simulink model "voltage_to_current_signal"  (R2024a)
settings: Solver=VariableStepAuto  StartTime=0.0  StopTime=0.1  RelTol=1e-3
libraries: fl_lib x93, nesl_utility x24
settings Model: Creator=ltnbda  LastModifiedBy=ltnbda
settings RTWCC: GPUComputeCapability=3.5

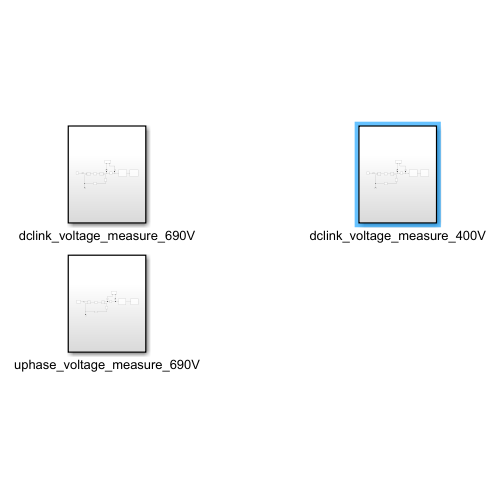
[thumbnail: Simulink's stored preview of the top-level diagram]
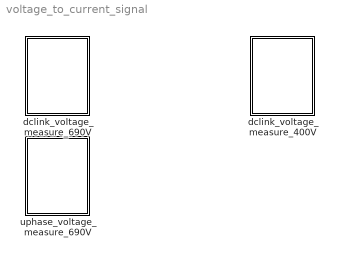
== system voltage_to_current_signal ==
  dclink_voltage_measure_400V : Subsystem
  dclink_voltage_measure_690V : Subsystem
  uphase_voltage_measure_690V : Subsystem

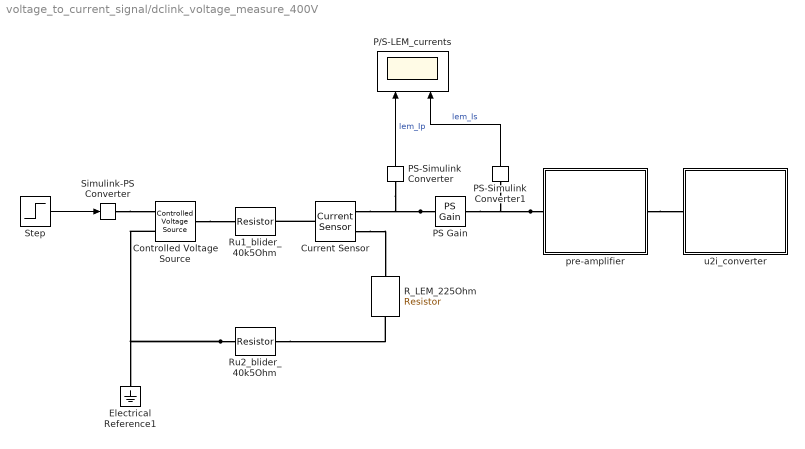
== system voltage_to_current_signal/dclink_voltage_measure_400V ==
  Controlled Voltage Source : fl_lib/Electrical/Electrical Sources/Controlled Voltage Source
  Current Sensor : fl_lib/Electrical/Electrical Sensors/Current Sensor
  Electrical Reference1 : fl_lib/Electrical/Electrical Elements/Electrical Reference
  P/S-LEM_currents : Scope  NumInputPorts=2
  PS Gain : fl_lib/Physical Signals/Functions/PS Gain  gain=2.5
  PS-Simulink Converter : nesl_utility/PS-Simulink Converter  PhysicalDomain=network_engine_domain  SubClassName=ps_output  LeftPortType=input  RightPortType=output  PseudoPeriodic=off  Frequencies=[]  VectorFormat=1-D array  Unit=A  AffineConversion=off
  PS-Simulink Converter1 : nesl_utility/PS-Simulink Converter  PhysicalDomain=network_engine_domain  SubClassName=ps_output  LeftPortType=input  RightPortType=output  PseudoPeriodic=off  Frequencies=[]  VectorFormat=1-D array  Unit=A  AffineConversion=off
  R_LEM_225Ohm : fl_lib/Electrical/Electrical Elements/Resistor  R=225 Ohm  i_specify=off  i_priority=None  i=0 A  i_nominal_specify=off  i_nominal_value=1  i_nominal_unit=A  v_specify=off  v_priority=None  v=0 V  v_nominal_specify=off  v_nominal_value=1  v_nominal_unit=V
  Ru1_blider_40k5Ohm : fl_lib/Electrical/Electrical Elements/Resistor  R=40.5e3 Ohm  i_specify=off  i_priority=None  i=0 A  i_nominal_specify=off  i_nominal_value=1  i_nominal_unit=A  v_specify=off  v_priority=None  v=0 V  v_nominal_specify=off  v_nominal_value=1  v_nominal_unit=V
  Ru2_blider_40k5Ohm : fl_lib/Electrical/Electrical Elements/Resistor  R=40.5e3 Ohm  i_specify=off  i_priority=None  i=0 A  i_nominal_specify=off  i_nominal_value=1  i_nominal_unit=A  v_specify=off  v_priority=None  v=0 V  v_nominal_specify=off  v_nominal_value=1  v_nominal_unit=V
  Simulink-PS Converter : nesl_utility/Simulink-PS Converter  PhysicalDomain=network_engine_domain  SubClassName=ps_input  LeftPortType=input  RightPortType=output  PseudoPeriodic=off  Frequencies=[]  NoiseDistribution=none  NoiseParameters=[]  Unit=V  AffineConversion=off  FilteringAndDerivatives=provide  SimscapeFilterOrder=1  InputFilterTimeConstant=0.001  UdotUserProvided=0
  Step : Step  Time=0.02  After=1000  SampleTime=0
  pre-amplifier : Subsystem
  u2i_converter : Subsystem
  wires:
  PS-Simulink Converter1/1 -> P/S-LEM_currents/2  "lem_Is"
  PS-Simulink Converter/1 -> P/S-LEM_currents/1  "lem_Ip"
  Step/1 -> Simulink-PS Converter/1
  connections:
  PS Gain/LConn1 -- PS-Simulink Converter/LConn1 -- Current Sensor/RConn1
  pre-amplifier/RConn1 -- u2i_converter/LConn1
  pre-amplifier/LConn1 -- PS-Simulink Converter1/LConn1 -- PS Gain/RConn1
  Current Sensor/RConn2 -- R_LEM_225Ohm/LConn1
  Current Sensor/LConn1 -- Ru1_blider_40k5Ohm/RConn1
  Ru2_blider_40k5Ohm/LConn1 -- Electrical Reference1/LConn1 -- Controlled Voltage Source/RConn2
  Controlled Voltage Source/LConn1 -- Ru1_blider_40k5Ohm/LConn1
  Ru2_blider_40k5Ohm/RConn1 -- R_LEM_225Ohm/RConn1
  Simulink-PS Converter/RConn1 -- Controlled Voltage Source/RConn1

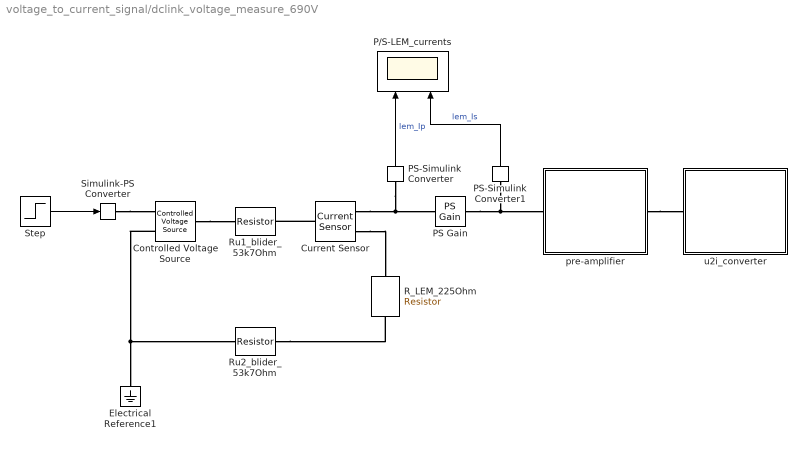
== system voltage_to_current_signal/dclink_voltage_measure_690V ==
  Controlled Voltage Source : fl_lib/Electrical/Electrical Sources/Controlled Voltage Source
  Current Sensor : fl_lib/Electrical/Electrical Sensors/Current Sensor
  Electrical Reference1 : fl_lib/Electrical/Electrical Elements/Electrical Reference
  P/S-LEM_currents : Scope  NumInputPorts=2
  PS Gain : fl_lib/Physical Signals/Functions/PS Gain  gain=2.5
  PS-Simulink Converter : nesl_utility/PS-Simulink Converter  PhysicalDomain=network_engine_domain  SubClassName=ps_output  LeftPortType=input  RightPortType=output  PseudoPeriodic=off  Frequencies=[]  VectorFormat=1-D array  Unit=A  AffineConversion=off
  PS-Simulink Converter1 : nesl_utility/PS-Simulink Converter  PhysicalDomain=network_engine_domain  SubClassName=ps_output  LeftPortType=input  RightPortType=output  PseudoPeriodic=off  Frequencies=[]  VectorFormat=1-D array  Unit=A  AffineConversion=off
  R_LEM_225Ohm : fl_lib/Electrical/Electrical Elements/Resistor  R=225 Ohm  i_specify=off  i_priority=None  i=0 A  i_nominal_specify=off  i_nominal_value=1  i_nominal_unit=A  v_specify=off  v_priority=None  v=0 V  v_nominal_specify=off  v_nominal_value=1  v_nominal_unit=V
  Ru1_blider_53k7Ohm : fl_lib/Electrical/Electrical Elements/Resistor  R=53.7e3 Ohm  i_specify=off  i_priority=None  i=0 A  i_nominal_specify=off  i_nominal_value=1  i_nominal_unit=A  v_specify=off  v_priority=None  v=0 V  v_nominal_specify=off  v_nominal_value=1  v_nominal_unit=V
  Ru2_blider_53k7Ohm : fl_lib/Electrical/Electrical Elements/Resistor  R=53.7e3 Ohm  i_specify=off  i_priority=None  i=0 A  i_nominal_specify=off  i_nominal_value=1  i_nominal_unit=A  v_specify=off  v_priority=None  v=0 V  v_nominal_specify=off  v_nominal_value=1  v_nominal_unit=V
  Simulink-PS Converter : nesl_utility/Simulink-PS Converter  PhysicalDomain=network_engine_domain  SubClassName=ps_input  LeftPortType=input  RightPortType=output  PseudoPeriodic=off  Frequencies=[]  NoiseDistribution=none  NoiseParameters=[]  Unit=V  AffineConversion=off  FilteringAndDerivatives=provide  SimscapeFilterOrder=1  InputFilterTimeConstant=0.001  UdotUserProvided=0
  Step : Step  Time=0.02  After=1500  SampleTime=0
  pre-amplifier : Subsystem
  u2i_converter : Subsystem
  wires:
  Step/1 -> Simulink-PS Converter/1
  PS-Simulink Converter/1 -> P/S-LEM_currents/1  "lem_Ip"
  PS-Simulink Converter1/1 -> P/S-LEM_currents/2  "lem_Is"
  connections:
  Simulink-PS Converter/RConn1 -- Controlled Voltage Source/RConn1
  Ru2_blider_53k7Ohm/RConn1 -- R_LEM_225Ohm/RConn1
  Controlled Voltage Source/LConn1 -- Ru1_blider_53k7Ohm/LConn1
  Controlled Voltage Source/RConn2 -- Electrical Reference1/LConn1 -- Ru2_blider_53k7Ohm/LConn1
  Current Sensor/LConn1 -- Ru1_blider_53k7Ohm/RConn1
  Current Sensor/RConn2 -- R_LEM_225Ohm/LConn1
  PS Gain/RConn1 -- PS-Simulink Converter1/LConn1 -- pre-amplifier/LConn1
  pre-amplifier/RConn1 -- u2i_converter/LConn1
  Current Sensor/RConn1 -- PS-Simulink Converter/LConn1 -- PS Gain/LConn1

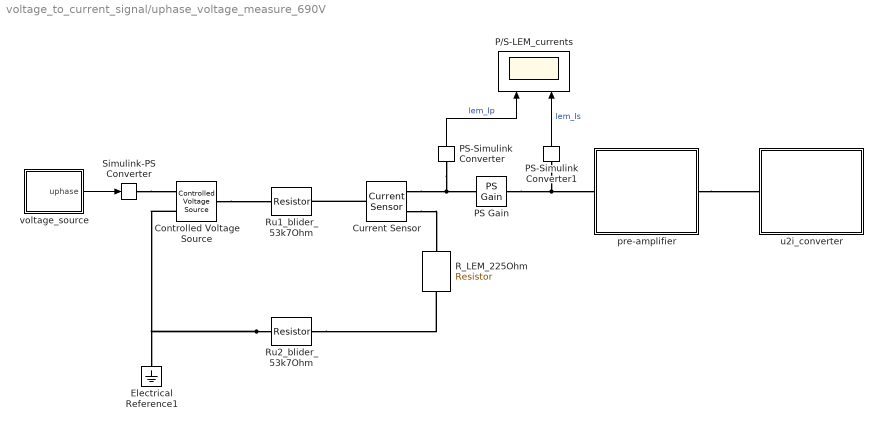
== system voltage_to_current_signal/uphase_voltage_measure_690V ==
  Controlled Voltage Source : fl_lib/Electrical/Electrical Sources/Controlled Voltage Source
  Current Sensor : fl_lib/Electrical/Electrical Sensors/Current Sensor
  Electrical Reference1 : fl_lib/Electrical/Electrical Elements/Electrical Reference
  P/S-LEM_currents : Scope  NumInputPorts=2
  PS Gain : fl_lib/Physical Signals/Functions/PS Gain  gain=2.5
  PS-Simulink Converter : nesl_utility/PS-Simulink Converter  PhysicalDomain=network_engine_domain  SubClassName=ps_output  LeftPortType=input  RightPortType=output  PseudoPeriodic=off  Frequencies=[]  VectorFormat=1-D array  Unit=A  AffineConversion=off
  PS-Simulink Converter1 : nesl_utility/PS-Simulink Converter  PhysicalDomain=network_engine_domain  SubClassName=ps_output  LeftPortType=input  RightPortType=output  PseudoPeriodic=off  Frequencies=[]  VectorFormat=1-D array  Unit=A  AffineConversion=off
  R_LEM_225Ohm : fl_lib/Electrical/Electrical Elements/Resistor  R=225 Ohm  i_specify=off  i_priority=None  i=0 A  i_nominal_specify=off  i_nominal_value=1  i_nominal_unit=A  v_specify=off  v_priority=None  v=0 V  v_nominal_specify=off  v_nominal_value=1  v_nominal_unit=V
  Ru1_blider_53k7Ohm : fl_lib/Electrical/Electrical Elements/Resistor  R=53.7e3 Ohm  i_specify=off  i_priority=None  i=0 A  i_nominal_specify=off  i_nominal_value=1  i_nominal_unit=A  v_specify=off  v_priority=None  v=0 V  v_nominal_specify=off  v_nominal_value=1  v_nominal_unit=V
  Ru2_blider_53k7Ohm : fl_lib/Electrical/Electrical Elements/Resistor  R=53.7e3 Ohm  i_specify=off  i_priority=None  i=0 A  i_nominal_specify=off  i_nominal_value=1  i_nominal_unit=A  v_specify=off  v_priority=None  v=0 V  v_nominal_specify=off  v_nominal_value=1  v_nominal_unit=V
  Simulink-PS Converter : nesl_utility/Simulink-PS Converter  PhysicalDomain=network_engine_domain  SubClassName=ps_input  LeftPortType=input  RightPortType=output  PseudoPeriodic=off  Frequencies=[]  NoiseDistribution=none  NoiseParameters=[]  Unit=V  AffineConversion=off  FilteringAndDerivatives=provide  SimscapeFilterOrder=1  InputFilterTimeConstant=0.001  UdotUserProvided=0
  pre-amplifier : Subsystem
  u2i_converter : Subsystem
  voltage_source : Subsystem
  wires:
  PS-Simulink Converter1/1 -> P/S-LEM_currents/2  "lem_Is"
  PS-Simulink Converter/1 -> P/S-LEM_currents/1  "lem_Ip"
  voltage_source/1(uphase) -> Simulink-PS Converter/1
  connections:
  PS-Simulink Converter/LConn1 -- Current Sensor/RConn1 -- PS Gain/LConn1
  pre-amplifier/RConn1 -- u2i_converter/LConn1
  PS-Simulink Converter1/LConn1 -- PS Gain/RConn1 -- pre-amplifier/LConn1
  Current Sensor/RConn2 -- R_LEM_225Ohm/LConn1
  Current Sensor/LConn1 -- Ru1_blider_53k7Ohm/RConn1
  Ru2_blider_53k7Ohm/LConn1 -- Electrical Reference1/LConn1 -- Controlled Voltage Source/RConn2
  Controlled Voltage Source/LConn1 -- Ru1_blider_53k7Ohm/LConn1
  Ru2_blider_53k7Ohm/RConn1 -- R_LEM_225Ohm/RConn1
  Simulink-PS Converter/RConn1 -- Controlled Voltage Source/RConn1

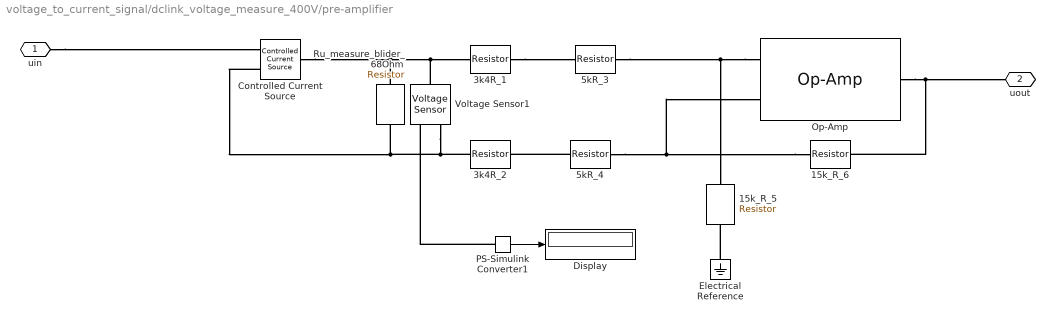
== system voltage_to_current_signal/dclink_voltage_measure_400V/pre-amplifier ==
  15k_R_5 : fl_lib/Electrical/Electrical Elements/Resistor  R=15e3 Ohm  i_specify=off  i_priority=None  i=0 A  i_nominal_specify=off  i_nominal_value=1  i_nominal_unit=A  v_specify=off  v_priority=None  v=0 V  v_nominal_specify=off  v_nominal_value=1  v_nominal_unit=V
  15k_R_6 : fl_lib/Electrical/Electrical Elements/Resistor  R=15e3 Ohm  i_specify=off  i_priority=None  i=0 A  i_nominal_specify=off  i_nominal_value=1  i_nominal_unit=A  v_specify=off  v_priority=None  v=0 V  v_nominal_specify=off  v_nominal_value=1  v_nominal_unit=V
  3k4R_1 : fl_lib/Electrical/Electrical Elements/Resistor  R=3.4e3 Ohm  i_specify=off  i_priority=None  i=0 A  i_nominal_specify=off  i_nominal_value=1  i_nominal_unit=A  v_specify=off  v_priority=None  v=0 V  v_nominal_specify=off  v_nominal_value=1  v_nominal_unit=V
  3k4R_2 : fl_lib/Electrical/Electrical Elements/Resistor  R=3.4e3 Ohm  i_specify=off  i_priority=None  i=0 A  i_nominal_specify=off  i_nominal_value=1  i_nominal_unit=A  v_specify=off  v_priority=None  v=0 V  v_nominal_specify=off  v_nominal_value=1  v_nominal_unit=V
  5kR_3 : fl_lib/Electrical/Electrical Elements/Resistor  R=5e3 Ohm  i_specify=off  i_priority=None  i=0 A  i_nominal_specify=off  i_nominal_value=1  i_nominal_unit=A  v_specify=off  v_priority=None  v=0 V  v_nominal_specify=off  v_nominal_value=1  v_nominal_unit=V
  5kR_4 : fl_lib/Electrical/Electrical Elements/Resistor  R=5e3 Ohm  i_specify=off  i_priority=None  i=0 A  i_nominal_specify=off  i_nominal_value=1  i_nominal_unit=A  v_specify=off  v_priority=None  v=0 V  v_nominal_specify=off  v_nominal_value=1  v_nominal_unit=V
  Controlled Current Source : fl_lib/Electrical/Electrical Sources/Controlled Current Source
  Display : Display
  Electrical Reference : fl_lib/Electrical/Electrical Elements/Electrical Reference
  Op-Amp : fl_lib/Electrical/Electrical Elements/Op-Amp  outI_specify=off  outI_priority=None  outI=0 A  outI_nominal_specify=off  outI_nominal_value=1  outI_nominal_unit=A
  PS-Simulink Converter1 : nesl_utility/PS-Simulink Converter  PhysicalDomain=network_engine_domain  SubClassName=ps_output  LeftPortType=input  RightPortType=output  PseudoPeriodic=off  Frequencies=[]  VectorFormat=1-D array  Unit=V  AffineConversion=off
  Ru_measure_blider_68Ohm : fl_lib/Electrical/Electrical Elements/Resistor  R=68 Ohm  i_specify=off  i_priority=None  i=0 A  i_nominal_specify=off  i_nominal_value=1  i_nominal_unit=A  v_specify=off  v_priority=None  v=0 V  v_nominal_specify=off  v_nominal_value=1  v_nominal_unit=V
  Voltage Sensor1 : fl_lib/Electrical/Electrical Sensors/Voltage Sensor
  uin : PMIOPort  Side=Left
  uout : PMIOPort  Port=2  Side=Right
  wires:
  PS-Simulink Converter1/1 -> Display/1
  connections:
  PS-Simulink Converter1/LConn1 -- Voltage Sensor1/RConn1
  uin/RConn1 -- Controlled Current Source/RConn1
  Ru_measure_blider_68Ohm/RConn1 -- Controlled Current Source/RConn2 -- Voltage Sensor1/RConn2 -- 3k4R_2/LConn1
  Controlled Current Source/LConn1 -- Voltage Sensor1/LConn1 -- 3k4R_1/LConn1 -- Ru_measure_blider_68Ohm/LConn1
  15k_R_6/LConn1 -- uout/RConn1 -- Op-Amp/RConn1
  15k_R_6/RConn1 -- Op-Amp/LConn2 -- 5kR_4/RConn1
  Op-Amp/LConn1 -- 15k_R_5/LConn1 -- 5kR_3/RConn1
  Electrical Reference/LConn1 -- 15k_R_5/RConn1
  5kR_4/LConn1 -- 3k4R_2/RConn1
  3k4R_1/RConn1 -- 5kR_3/LConn1

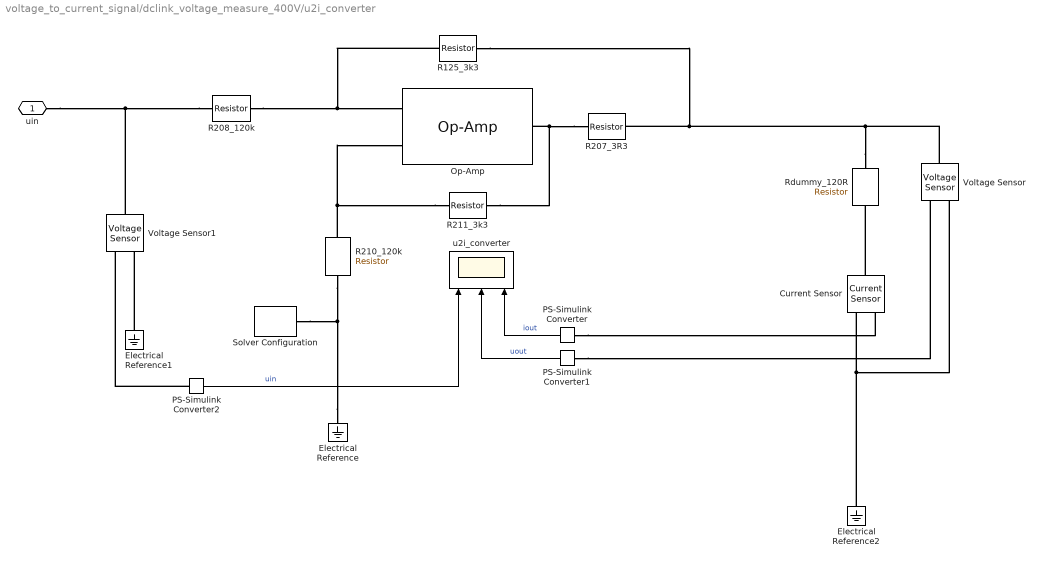
== system voltage_to_current_signal/dclink_voltage_measure_400V/u2i_converter ==
  Current Sensor : fl_lib/Electrical/Electrical Sensors/Current Sensor
  Electrical Reference : fl_lib/Electrical/Electrical Elements/Electrical Reference
  Electrical Reference1 : fl_lib/Electrical/Electrical Elements/Electrical Reference
  Electrical Reference2 : fl_lib/Electrical/Electrical Elements/Electrical Reference
  Op-Amp : fl_lib/Electrical/Electrical Elements/Op-Amp  outI_specify=off  outI_priority=None  outI=0 A  outI_nominal_specify=off  outI_nominal_value=1  outI_nominal_unit=A
  PS-Simulink Converter : nesl_utility/PS-Simulink Converter  PhysicalDomain=network_engine_domain  SubClassName=ps_output  LeftPortType=input  RightPortType=output  PseudoPeriodic=off  Frequencies=[]  VectorFormat=1-D array  Unit=A  AffineConversion=off
  PS-Simulink Converter1 : nesl_utility/PS-Simulink Converter  PhysicalDomain=network_engine_domain  SubClassName=ps_output  LeftPortType=input  RightPortType=output  PseudoPeriodic=off  Frequencies=[]  VectorFormat=1-D array  Unit=V  AffineConversion=off
  PS-Simulink Converter2 : nesl_utility/PS-Simulink Converter  PhysicalDomain=network_engine_domain  SubClassName=ps_output  LeftPortType=input  RightPortType=output  PseudoPeriodic=off  Frequencies=[]  VectorFormat=1-D array  Unit=V  AffineConversion=off
  R125_3k3 : fl_lib/Electrical/Electrical Elements/Resistor  R=3.3e3 Ohm  i_specify=off  i_priority=None  i=0 A  i_nominal_specify=off  i_nominal_value=1  i_nominal_unit=A  v_specify=off  v_priority=None  v=0 V  v_nominal_specify=off  v_nominal_value=1  v_nominal_unit=V
  R207_3R3 : fl_lib/Electrical/Electrical Elements/Resistor  R=3.3 Ohm  i_specify=off  i_priority=None  i=0 A  i_nominal_specify=off  i_nominal_value=1  i_nominal_unit=A  v_specify=off  v_priority=None  v=0 V  v_nominal_specify=off  v_nominal_value=1  v_nominal_unit=V
  R208_120k : fl_lib/Electrical/Electrical Elements/Resistor  R=120e3 Ohm  i_specify=off  i_priority=None  i=0 A  i_nominal_specify=off  i_nominal_value=1  i_nominal_unit=A  v_specify=off  v_priority=None  v=0 V  v_nominal_specify=off  v_nominal_value=1  v_nominal_unit=V
  R210_120k : fl_lib/Electrical/Electrical Elements/Resistor  R=120e3 Ohm  i_specify=off  i_priority=None  i=0 A  i_nominal_specify=off  i_nominal_value=1  i_nominal_unit=A  v_specify=off  v_priority=None  v=0 V  v_nominal_specify=off  v_nominal_value=1  v_nominal_unit=V
  R211_3k3 : fl_lib/Electrical/Electrical Elements/Resistor  R=3.3e3 Ohm  i_specify=off  i_priority=None  i=0 A  i_nominal_specify=off  i_nominal_value=1  i_nominal_unit=A  v_specify=off  v_priority=None  v=0 V  v_nominal_specify=off  v_nominal_value=1  v_nominal_unit=V
  Rdummy_120R : fl_lib/Electrical/Electrical Elements/Resistor  R=120 Ohm  i_specify=off  i_priority=None  i=0 A  i_nominal_specify=off  i_nominal_value=1  i_nominal_unit=A  v_specify=off  v_priority=None  v=0 V  v_nominal_specify=off  v_nominal_value=1  v_nominal_unit=V
  Solver Configuration : nesl_utility/Solver Configuration  PhysicalDomain=network_engine_domain  SubClassName=solver  LeftPortType=input  RightPortType=generic  Tones=[]  Harmonics=[]  SimulateNoise=off  Profile=off  UseLocalSampling=off  EnableSwitchedLinearOptims=on  FrequencyDomain=off  UseCCode=off  RelTol=0.001  AbsTol=0.001  MinStep=1e-09  ToWorkspace=off  RevertToSquareIcSolve=off  NumHomotopyIterations=100  PhasorMode=off  PhasorModeNumHarmonics=1  ConsistencySolver=NEWTON_XTOL_AFTER_FTOL  IndexReductionMethod=DerivativeReplacement  DoDC=on  ResidualTolerance=1e-09  ConsistencyTolSource=GLOBAL  ConsistencyAbsTol=0.001  ConsistencyRelTol=0.001  ConsistencyTolFactor=0.001  UseLocalSolver=on  LocalSolverChoice=NE_BACKWARD_EULER_ADVANCER  ResolveIndetEquations=on  FunctionEvalNumThread=1  LocalSolverSampleTime=1e-6  DoFixedCost=on  MaxNonlinIter=3  MaxModeIter=2  ComputeImpulses=off  ImpulseIterations=2  LinearAlgebra=auto  LinearAlgebraNumThread=0  EquationFormulation=NE_TIME_EF  DelaysMemoryBudget=1024  AutomaticFiltering=on  FilteringTimeConstant=0.001  PartitionStorageMethod=AS_NEEDED  PartitionMemoryBudget=1024  PartitionMethod=ROBUST  MultibodyUseLocalSolver=off  MultibodyLocalSolverChoice=ODE1  MultibodyLocalSolverSampleTime=0.001
  Voltage Sensor : fl_lib/Electrical/Electrical Sensors/Voltage Sensor
  Voltage Sensor1 : fl_lib/Electrical/Electrical Sensors/Voltage Sensor
  u2i_converter : Scope  NumInputPorts=3
  uin : PMIOPort  Side=Left
  wires:
  PS-Simulink Converter2/1 -> u2i_converter/1  "uin"
  PS-Simulink Converter/1 -> u2i_converter/3  "iout"
  PS-Simulink Converter1/1 -> u2i_converter/2  "uout"
  connections:
  PS-Simulink Converter2/LConn1 -- Voltage Sensor1/RConn1
  Electrical Reference1/LConn1 -- Voltage Sensor1/RConn2
  PS-Simulink Converter1/LConn1 -- Voltage Sensor/RConn1
  R208_120k/LConn1 -- Voltage Sensor1/LConn1 -- uin/RConn1
  Rdummy_120R/LConn1 -- R207_3R3/RConn1 -- R125_3k3/RConn1 -- Voltage Sensor/LConn1
  PS-Simulink Converter/LConn1 -- Current Sensor/RConn1
  Current Sensor/LConn1 -- Rdummy_120R/RConn1
  Electrical Reference/LConn1 -- Solver Configuration/RConn1 -- R210_120k/RConn1
  R211_3k3/LConn1 -- Op-Amp/LConn2 -- R210_120k/LConn1
  R125_3k3/LConn1 -- Op-Amp/LConn1 -- R208_120k/RConn1
  Current Sensor/RConn2 -- Voltage Sensor/RConn2 -- Electrical Reference2/LConn1
  R207_3R3/LConn1 -- Op-Amp/RConn1 -- R211_3k3/RConn1

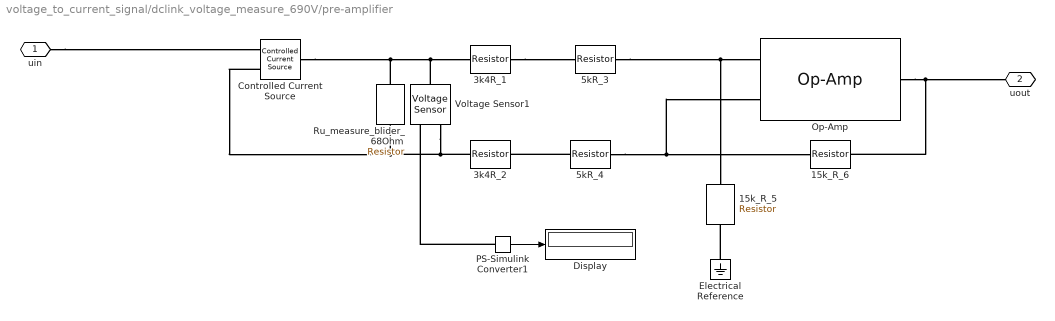
== system voltage_to_current_signal/dclink_voltage_measure_690V/pre-amplifier ==
  15k_R_5 : fl_lib/Electrical/Electrical Elements/Resistor  R=15e3 Ohm  i_specify=off  i_priority=None  i=0 A  i_nominal_specify=off  i_nominal_value=1  i_nominal_unit=A  v_specify=off  v_priority=None  v=0 V  v_nominal_specify=off  v_nominal_value=1  v_nominal_unit=V
  15k_R_6 : fl_lib/Electrical/Electrical Elements/Resistor  R=15e3 Ohm  i_specify=off  i_priority=None  i=0 A  i_nominal_specify=off  i_nominal_value=1  i_nominal_unit=A  v_specify=off  v_priority=None  v=0 V  v_nominal_specify=off  v_nominal_value=1  v_nominal_unit=V
  3k4R_1 : fl_lib/Electrical/Electrical Elements/Resistor  R=3.4e3 Ohm  i_specify=off  i_priority=None  i=0 A  i_nominal_specify=off  i_nominal_value=1  i_nominal_unit=A  v_specify=off  v_priority=None  v=0 V  v_nominal_specify=off  v_nominal_value=1  v_nominal_unit=V
  3k4R_2 : fl_lib/Electrical/Electrical Elements/Resistor  R=3.4e3 Ohm  i_specify=off  i_priority=None  i=0 A  i_nominal_specify=off  i_nominal_value=1  i_nominal_unit=A  v_specify=off  v_priority=None  v=0 V  v_nominal_specify=off  v_nominal_value=1  v_nominal_unit=V
  5kR_3 : fl_lib/Electrical/Electrical Elements/Resistor  R=5e3 Ohm  i_specify=off  i_priority=None  i=0 A  i_nominal_specify=off  i_nominal_value=1  i_nominal_unit=A  v_specify=off  v_priority=None  v=0 V  v_nominal_specify=off  v_nominal_value=1  v_nominal_unit=V
  5kR_4 : fl_lib/Electrical/Electrical Elements/Resistor  R=5e3 Ohm  i_specify=off  i_priority=None  i=0 A  i_nominal_specify=off  i_nominal_value=1  i_nominal_unit=A  v_specify=off  v_priority=None  v=0 V  v_nominal_specify=off  v_nominal_value=1  v_nominal_unit=V
  Controlled Current Source : fl_lib/Electrical/Electrical Sources/Controlled Current Source
  Display : Display
  Electrical Reference : fl_lib/Electrical/Electrical Elements/Electrical Reference
  Op-Amp : fl_lib/Electrical/Electrical Elements/Op-Amp  outI_specify=off  outI_priority=None  outI=0 A  outI_nominal_specify=off  outI_nominal_value=1  outI_nominal_unit=A
  PS-Simulink Converter1 : nesl_utility/PS-Simulink Converter  PhysicalDomain=network_engine_domain  SubClassName=ps_output  LeftPortType=input  RightPortType=output  PseudoPeriodic=off  Frequencies=[]  VectorFormat=1-D array  Unit=V  AffineConversion=off
  Ru_measure_blider_68Ohm : fl_lib/Electrical/Electrical Elements/Resistor  R=68 Ohm  i_specify=off  i_priority=None  i=0 A  i_nominal_specify=off  i_nominal_value=1  i_nominal_unit=A  v_specify=off  v_priority=None  v=0 V  v_nominal_specify=off  v_nominal_value=1  v_nominal_unit=V
  Voltage Sensor1 : fl_lib/Electrical/Electrical Sensors/Voltage Sensor
  uin : PMIOPort  Side=Left
  uout : PMIOPort  Port=2  Side=Right
  wires:
  PS-Simulink Converter1/1 -> Display/1
  connections:
  3k4R_1/RConn1 -- 5kR_3/LConn1
  5kR_4/LConn1 -- 3k4R_2/RConn1
  Electrical Reference/LConn1 -- 15k_R_5/RConn1
  5kR_3/RConn1 -- 15k_R_5/LConn1 -- Op-Amp/LConn1
  5kR_4/RConn1 -- Op-Amp/LConn2 -- 15k_R_6/RConn1
  Op-Amp/RConn1 -- uout/RConn1 -- 15k_R_6/LConn1
  Ru_measure_blider_68Ohm/LConn1 -- 3k4R_1/LConn1 -- Voltage Sensor1/LConn1 -- Controlled Current Source/LConn1
  3k4R_2/LConn1 -- Voltage Sensor1/RConn2 -- Controlled Current Source/RConn2 -- Ru_measure_blider_68Ohm/RConn1
  uin/RConn1 -- Controlled Current Source/RConn1
  PS-Simulink Converter1/LConn1 -- Voltage Sensor1/RConn1

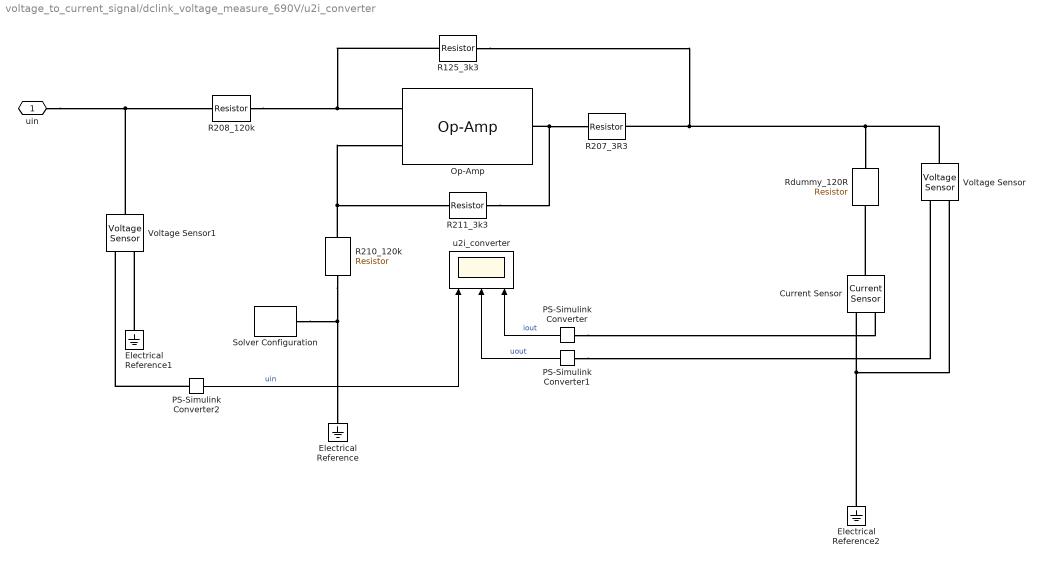
== system voltage_to_current_signal/dclink_voltage_measure_690V/u2i_converter ==
  Current Sensor : fl_lib/Electrical/Electrical Sensors/Current Sensor
  Electrical Reference : fl_lib/Electrical/Electrical Elements/Electrical Reference
  Electrical Reference1 : fl_lib/Electrical/Electrical Elements/Electrical Reference
  Electrical Reference2 : fl_lib/Electrical/Electrical Elements/Electrical Reference
  Op-Amp : fl_lib/Electrical/Electrical Elements/Op-Amp  outI_specify=off  outI_priority=None  outI=0 A  outI_nominal_specify=off  outI_nominal_value=1  outI_nominal_unit=A
  PS-Simulink Converter : nesl_utility/PS-Simulink Converter  PhysicalDomain=network_engine_domain  SubClassName=ps_output  LeftPortType=input  RightPortType=output  PseudoPeriodic=off  Frequencies=[]  VectorFormat=1-D array  Unit=A  AffineConversion=off
  PS-Simulink Converter1 : nesl_utility/PS-Simulink Converter  PhysicalDomain=network_engine_domain  SubClassName=ps_output  LeftPortType=input  RightPortType=output  PseudoPeriodic=off  Frequencies=[]  VectorFormat=1-D array  Unit=V  AffineConversion=off
  PS-Simulink Converter2 : nesl_utility/PS-Simulink Converter  PhysicalDomain=network_engine_domain  SubClassName=ps_output  LeftPortType=input  RightPortType=output  PseudoPeriodic=off  Frequencies=[]  VectorFormat=1-D array  Unit=V  AffineConversion=off
  R125_3k3 : fl_lib/Electrical/Electrical Elements/Resistor  R=3.3e3 Ohm  i_specify=off  i_priority=None  i=0 A  i_nominal_specify=off  i_nominal_value=1  i_nominal_unit=A  v_specify=off  v_priority=None  v=0 V  v_nominal_specify=off  v_nominal_value=1  v_nominal_unit=V
  R207_3R3 : fl_lib/Electrical/Electrical Elements/Resistor  R=3.3 Ohm  i_specify=off  i_priority=None  i=0 A  i_nominal_specify=off  i_nominal_value=1  i_nominal_unit=A  v_specify=off  v_priority=None  v=0 V  v_nominal_specify=off  v_nominal_value=1  v_nominal_unit=V
  R208_120k : fl_lib/Electrical/Electrical Elements/Resistor  R=120e3 Ohm  i_specify=off  i_priority=None  i=0 A  i_nominal_specify=off  i_nominal_value=1  i_nominal_unit=A  v_specify=off  v_priority=None  v=0 V  v_nominal_specify=off  v_nominal_value=1  v_nominal_unit=V
  R210_120k : fl_lib/Electrical/Electrical Elements/Resistor  R=120e3 Ohm  i_specify=off  i_priority=None  i=0 A  i_nominal_specify=off  i_nominal_value=1  i_nominal_unit=A  v_specify=off  v_priority=None  v=0 V  v_nominal_specify=off  v_nominal_value=1  v_nominal_unit=V
  R211_3k3 : fl_lib/Electrical/Electrical Elements/Resistor  R=3.3e3 Ohm  i_specify=off  i_priority=None  i=0 A  i_nominal_specify=off  i_nominal_value=1  i_nominal_unit=A  v_specify=off  v_priority=None  v=0 V  v_nominal_specify=off  v_nominal_value=1  v_nominal_unit=V
  Rdummy_120R : fl_lib/Electrical/Electrical Elements/Resistor  R=120 Ohm  i_specify=off  i_priority=None  i=0 A  i_nominal_specify=off  i_nominal_value=1  i_nominal_unit=A  v_specify=off  v_priority=None  v=0 V  v_nominal_specify=off  v_nominal_value=1  v_nominal_unit=V
  Solver Configuration : nesl_utility/Solver Configuration  PhysicalDomain=network_engine_domain  SubClassName=solver  LeftPortType=input  RightPortType=generic  Tones=[]  Harmonics=[]  SimulateNoise=off  Profile=off  UseLocalSampling=off  EnableSwitchedLinearOptims=on  FrequencyDomain=off  UseCCode=off  RelTol=0.001  AbsTol=0.001  MinStep=1e-09  ToWorkspace=off  RevertToSquareIcSolve=off  NumHomotopyIterations=100  PhasorMode=off  PhasorModeNumHarmonics=1  ConsistencySolver=NEWTON_XTOL_AFTER_FTOL  IndexReductionMethod=DerivativeReplacement  DoDC=on  ResidualTolerance=1e-09  ConsistencyTolSource=GLOBAL  ConsistencyAbsTol=0.001  ConsistencyRelTol=0.001  ConsistencyTolFactor=0.001  UseLocalSolver=on  LocalSolverChoice=NE_BACKWARD_EULER_ADVANCER  ResolveIndetEquations=on  FunctionEvalNumThread=1  LocalSolverSampleTime=1e-6  DoFixedCost=on  MaxNonlinIter=3  MaxModeIter=2  ComputeImpulses=off  ImpulseIterations=2  LinearAlgebra=auto  LinearAlgebraNumThread=0  EquationFormulation=NE_TIME_EF  DelaysMemoryBudget=1024  AutomaticFiltering=on  FilteringTimeConstant=0.001  PartitionStorageMethod=AS_NEEDED  PartitionMemoryBudget=1024  PartitionMethod=ROBUST  MultibodyUseLocalSolver=off  MultibodyLocalSolverChoice=ODE1  MultibodyLocalSolverSampleTime=0.001
  Voltage Sensor : fl_lib/Electrical/Electrical Sensors/Voltage Sensor
  Voltage Sensor1 : fl_lib/Electrical/Electrical Sensors/Voltage Sensor
  u2i_converter : Scope  NumInputPorts=3
  uin : PMIOPort  Side=Left
  wires:
  PS-Simulink Converter1/1 -> u2i_converter/2  "uout"
  PS-Simulink Converter/1 -> u2i_converter/3  "iout"
  PS-Simulink Converter2/1 -> u2i_converter/1  "uin"
  connections:
  R211_3k3/RConn1 -- Op-Amp/RConn1 -- R207_3R3/LConn1
  Electrical Reference2/LConn1 -- Voltage Sensor/RConn2 -- Current Sensor/RConn2
  R208_120k/RConn1 -- Op-Amp/LConn1 -- R125_3k3/LConn1
  R210_120k/LConn1 -- Op-Amp/LConn2 -- R211_3k3/LConn1
  R210_120k/RConn1 -- Solver Configuration/RConn1 -- Electrical Reference/LConn1
  Current Sensor/LConn1 -- Rdummy_120R/RConn1
  PS-Simulink Converter/LConn1 -- Current Sensor/RConn1
  Voltage Sensor/LConn1 -- R125_3k3/RConn1 -- R207_3R3/RConn1 -- Rdummy_120R/LConn1
  uin/RConn1 -- Voltage Sensor1/LConn1 -- R208_120k/LConn1
  PS-Simulink Converter1/LConn1 -- Voltage Sensor/RConn1
  Electrical Reference1/LConn1 -- Voltage Sensor1/RConn2
  PS-Simulink Converter2/LConn1 -- Voltage Sensor1/RConn1

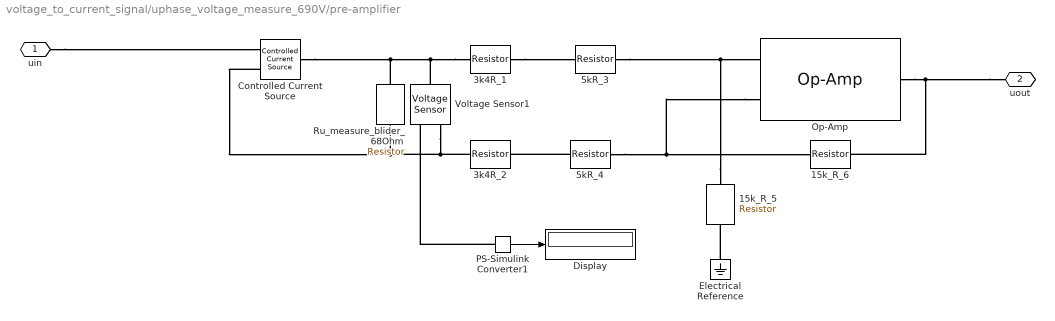
== system voltage_to_current_signal/uphase_voltage_measure_690V/pre-amplifier ==
  15k_R_5 : fl_lib/Electrical/Electrical Elements/Resistor  R=15e3 Ohm  i_specify=off  i_priority=None  i=0 A  i_nominal_specify=off  i_nominal_value=1  i_nominal_unit=A  v_specify=off  v_priority=None  v=0 V  v_nominal_specify=off  v_nominal_value=1  v_nominal_unit=V
  15k_R_6 : fl_lib/Electrical/Electrical Elements/Resistor  R=15e3 Ohm  i_specify=off  i_priority=None  i=0 A  i_nominal_specify=off  i_nominal_value=1  i_nominal_unit=A  v_specify=off  v_priority=None  v=0 V  v_nominal_specify=off  v_nominal_value=1  v_nominal_unit=V
  3k4R_1 : fl_lib/Electrical/Electrical Elements/Resistor  R=3.4e3 Ohm  i_specify=off  i_priority=None  i=0 A  i_nominal_specify=off  i_nominal_value=1  i_nominal_unit=A  v_specify=off  v_priority=None  v=0 V  v_nominal_specify=off  v_nominal_value=1  v_nominal_unit=V
  3k4R_2 : fl_lib/Electrical/Electrical Elements/Resistor  R=3.4e3 Ohm  i_specify=off  i_priority=None  i=0 A  i_nominal_specify=off  i_nominal_value=1  i_nominal_unit=A  v_specify=off  v_priority=None  v=0 V  v_nominal_specify=off  v_nominal_value=1  v_nominal_unit=V
  5kR_3 : fl_lib/Electrical/Electrical Elements/Resistor  R=5e3 Ohm  i_specify=off  i_priority=None  i=0 A  i_nominal_specify=off  i_nominal_value=1  i_nominal_unit=A  v_specify=off  v_priority=None  v=0 V  v_nominal_specify=off  v_nominal_value=1  v_nominal_unit=V
  5kR_4 : fl_lib/Electrical/Electrical Elements/Resistor  R=5e3 Ohm  i_specify=off  i_priority=None  i=0 A  i_nominal_specify=off  i_nominal_value=1  i_nominal_unit=A  v_specify=off  v_priority=None  v=0 V  v_nominal_specify=off  v_nominal_value=1  v_nominal_unit=V
  Controlled Current Source : fl_lib/Electrical/Electrical Sources/Controlled Current Source
  Display : Display
  Electrical Reference : fl_lib/Electrical/Electrical Elements/Electrical Reference
  Op-Amp : fl_lib/Electrical/Electrical Elements/Op-Amp  outI_specify=off  outI_priority=None  outI=0 A  outI_nominal_specify=off  outI_nominal_value=1  outI_nominal_unit=A
  PS-Simulink Converter1 : nesl_utility/PS-Simulink Converter  PhysicalDomain=network_engine_domain  SubClassName=ps_output  LeftPortType=input  RightPortType=output  PseudoPeriodic=off  Frequencies=[]  VectorFormat=1-D array  Unit=V  AffineConversion=off
  Ru_measure_blider_68Ohm : fl_lib/Electrical/Electrical Elements/Resistor  R=68 Ohm  i_specify=off  i_priority=None  i=0 A  i_nominal_specify=off  i_nominal_value=1  i_nominal_unit=A  v_specify=off  v_priority=None  v=0 V  v_nominal_specify=off  v_nominal_value=1  v_nominal_unit=V
  Voltage Sensor1 : fl_lib/Electrical/Electrical Sensors/Voltage Sensor
  uin : PMIOPort  Side=Left
  uout : PMIOPort  Port=2  Side=Right
  wires:
  PS-Simulink Converter1/1 -> Display/1
  connections:
  PS-Simulink Converter1/LConn1 -- Voltage Sensor1/RConn1
  uin/RConn1 -- Controlled Current Source/RConn1
  Voltage Sensor1/RConn2 -- Ru_measure_blider_68Ohm/RConn1 -- Controlled Current Source/RConn2 -- 3k4R_2/LConn1
  3k4R_1/LConn1 -- Voltage Sensor1/LConn1 -- Ru_measure_blider_68Ohm/LConn1 -- Controlled Current Source/LConn1
  uout/RConn1 -- 15k_R_6/LConn1 -- Op-Amp/RConn1
  Op-Amp/LConn2 -- 15k_R_6/RConn1 -- 5kR_4/RConn1
  15k_R_5/LConn1 -- Op-Amp/LConn1 -- 5kR_3/RConn1
  Electrical Reference/LConn1 -- 15k_R_5/RConn1
  5kR_4/LConn1 -- 3k4R_2/RConn1
  3k4R_1/RConn1 -- 5kR_3/LConn1

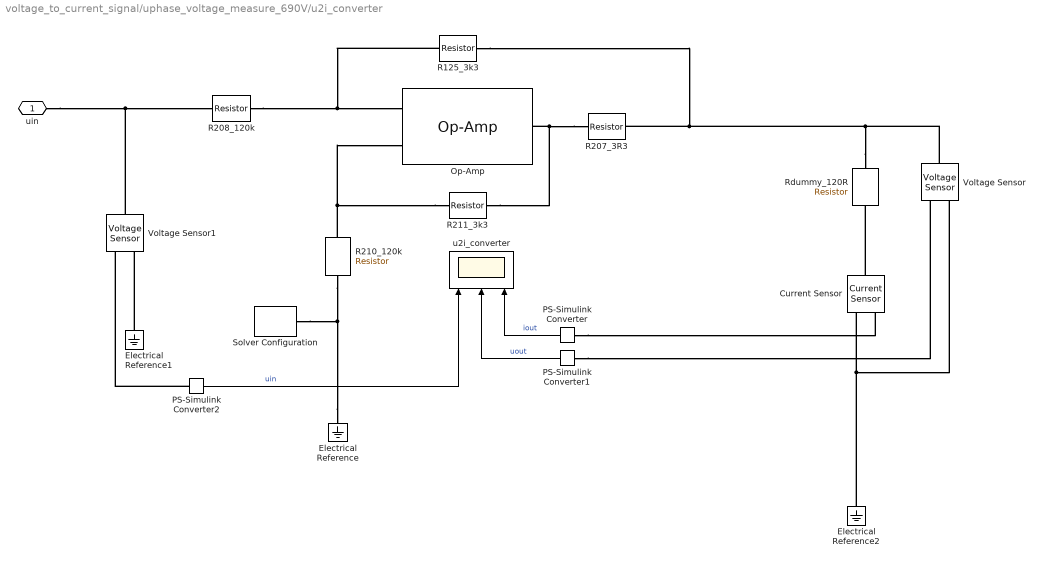
== system voltage_to_current_signal/uphase_voltage_measure_690V/u2i_converter ==
  Current Sensor : fl_lib/Electrical/Electrical Sensors/Current Sensor
  Electrical Reference : fl_lib/Electrical/Electrical Elements/Electrical Reference
  Electrical Reference1 : fl_lib/Electrical/Electrical Elements/Electrical Reference
  Electrical Reference2 : fl_lib/Electrical/Electrical Elements/Electrical Reference
  Op-Amp : fl_lib/Electrical/Electrical Elements/Op-Amp  outI_specify=off  outI_priority=None  outI=0 A  outI_nominal_specify=off  outI_nominal_value=1  outI_nominal_unit=A
  PS-Simulink Converter : nesl_utility/PS-Simulink Converter  PhysicalDomain=network_engine_domain  SubClassName=ps_output  LeftPortType=input  RightPortType=output  PseudoPeriodic=off  Frequencies=[]  VectorFormat=1-D array  Unit=A  AffineConversion=off
  PS-Simulink Converter1 : nesl_utility/PS-Simulink Converter  PhysicalDomain=network_engine_domain  SubClassName=ps_output  LeftPortType=input  RightPortType=output  PseudoPeriodic=off  Frequencies=[]  VectorFormat=1-D array  Unit=V  AffineConversion=off
  PS-Simulink Converter2 : nesl_utility/PS-Simulink Converter  PhysicalDomain=network_engine_domain  SubClassName=ps_output  LeftPortType=input  RightPortType=output  PseudoPeriodic=off  Frequencies=[]  VectorFormat=1-D array  Unit=V  AffineConversion=off
  R125_3k3 : fl_lib/Electrical/Electrical Elements/Resistor  R=3.3e3 Ohm  i_specify=off  i_priority=None  i=0 A  i_nominal_specify=off  i_nominal_value=1  i_nominal_unit=A  v_specify=off  v_priority=None  v=0 V  v_nominal_specify=off  v_nominal_value=1  v_nominal_unit=V
  R207_3R3 : fl_lib/Electrical/Electrical Elements/Resistor  R=3.3 Ohm  i_specify=off  i_priority=None  i=0 A  i_nominal_specify=off  i_nominal_value=1  i_nominal_unit=A  v_specify=off  v_priority=None  v=0 V  v_nominal_specify=off  v_nominal_value=1  v_nominal_unit=V
  R208_120k : fl_lib/Electrical/Electrical Elements/Resistor  R=120e3 Ohm  i_specify=off  i_priority=None  i=0 A  i_nominal_specify=off  i_nominal_value=1  i_nominal_unit=A  v_specify=off  v_priority=None  v=0 V  v_nominal_specify=off  v_nominal_value=1  v_nominal_unit=V
  R210_120k : fl_lib/Electrical/Electrical Elements/Resistor  R=120e3 Ohm  i_specify=off  i_priority=None  i=0 A  i_nominal_specify=off  i_nominal_value=1  i_nominal_unit=A  v_specify=off  v_priority=None  v=0 V  v_nominal_specify=off  v_nominal_value=1  v_nominal_unit=V
  R211_3k3 : fl_lib/Electrical/Electrical Elements/Resistor  R=3.3e3 Ohm  i_specify=off  i_priority=None  i=0 A  i_nominal_specify=off  i_nominal_value=1  i_nominal_unit=A  v_specify=off  v_priority=None  v=0 V  v_nominal_specify=off  v_nominal_value=1  v_nominal_unit=V
  Rdummy_120R : fl_lib/Electrical/Electrical Elements/Resistor  R=120 Ohm  i_specify=off  i_priority=None  i=0 A  i_nominal_specify=off  i_nominal_value=1  i_nominal_unit=A  v_specify=off  v_priority=None  v=0 V  v_nominal_specify=off  v_nominal_value=1  v_nominal_unit=V
  Solver Configuration : nesl_utility/Solver Configuration  PhysicalDomain=network_engine_domain  SubClassName=solver  LeftPortType=input  RightPortType=generic  Tones=[]  Harmonics=[]  SimulateNoise=off  Profile=off  UseLocalSampling=off  EnableSwitchedLinearOptims=on  FrequencyDomain=off  UseCCode=off  RelTol=0.001  AbsTol=0.001  MinStep=1e-09  ToWorkspace=off  RevertToSquareIcSolve=off  NumHomotopyIterations=100  PhasorMode=off  PhasorModeNumHarmonics=1  ConsistencySolver=NEWTON_XTOL_AFTER_FTOL  IndexReductionMethod=DerivativeReplacement  DoDC=on  ResidualTolerance=1e-09  ConsistencyTolSource=GLOBAL  ConsistencyAbsTol=0.001  ConsistencyRelTol=0.001  ConsistencyTolFactor=0.001  UseLocalSolver=on  LocalSolverChoice=NE_BACKWARD_EULER_ADVANCER  ResolveIndetEquations=on  FunctionEvalNumThread=1  LocalSolverSampleTime=1e-6  DoFixedCost=on  MaxNonlinIter=3  MaxModeIter=2  ComputeImpulses=off  ImpulseIterations=2  LinearAlgebra=auto  LinearAlgebraNumThread=0  EquationFormulation=NE_TIME_EF  DelaysMemoryBudget=1024  AutomaticFiltering=on  FilteringTimeConstant=0.001  PartitionStorageMethod=AS_NEEDED  PartitionMemoryBudget=1024  PartitionMethod=ROBUST  MultibodyUseLocalSolver=off  MultibodyLocalSolverChoice=ODE1  MultibodyLocalSolverSampleTime=0.001
  Voltage Sensor : fl_lib/Electrical/Electrical Sensors/Voltage Sensor
  Voltage Sensor1 : fl_lib/Electrical/Electrical Sensors/Voltage Sensor
  u2i_converter : Scope  NumInputPorts=3
  uin : PMIOPort  Side=Left
  wires:
  PS-Simulink Converter2/1 -> u2i_converter/1  "uin"
  PS-Simulink Converter/1 -> u2i_converter/3  "iout"
  PS-Simulink Converter1/1 -> u2i_converter/2  "uout"
  connections:
  PS-Simulink Converter2/LConn1 -- Voltage Sensor1/RConn1
  Electrical Reference1/LConn1 -- Voltage Sensor1/RConn2
  PS-Simulink Converter1/LConn1 -- Voltage Sensor/RConn1
  Voltage Sensor1/LConn1 -- uin/RConn1 -- R208_120k/LConn1
  Rdummy_120R/LConn1 -- R207_3R3/RConn1 -- R125_3k3/RConn1 -- Voltage Sensor/LConn1
  PS-Simulink Converter/LConn1 -- Current Sensor/RConn1
  Current Sensor/LConn1 -- Rdummy_120R/RConn1
  Electrical Reference/LConn1 -- Solver Configuration/RConn1 -- R210_120k/RConn1
  R211_3k3/LConn1 -- Op-Amp/LConn2 -- R210_120k/LConn1
  R125_3k3/LConn1 -- Op-Amp/LConn1 -- R208_120k/RConn1
  Current Sensor/RConn2 -- Voltage Sensor/RConn2 -- Electrical Reference2/LConn1
  R207_3R3/LConn1 -- Op-Amp/RConn1 -- R211_3k3/RConn1

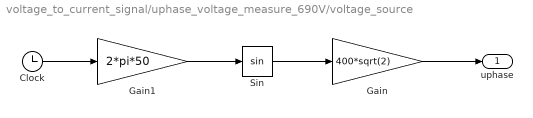
== system voltage_to_current_signal/uphase_voltage_measure_690V/voltage_source ==
  Clock : Clock
  Gain : Gain  Gain=400*sqrt(2)
  Gain1 : Gain  Gain=2*pi*50
  Sin : Trigonometry
  uphase : Outport
  wires:
  Gain/1 -> uphase/1
  Sin/1 -> Gain/1
  Gain1/1 -> Sin/1
  Clock/1 -> Gain1/1
